simulink model "mocp_simulink_block"  (R2016b)
settings: Solver=ode45  StartTime=0.0  StopTime=0.1  RelTol=1e-3
values from neighbouring files (symbols this model uses):
  ignore_inits = 0    [main_mocp_simulink.m]
  lbu_all = bu_fact * lbu_all    [main_mocp_simulink.m]
  lbx_all = [repmat(phase_1.constraints.lbx, N_list(1)-1, 1) ... (first row only)    [main_mocp_simulink.m]
  lh_all = [repmat(phase_1.constraints.lh, N_list(1)-1, 1) ... (first row only)    [main_mocp_simulink.m]
  pi_init = 0 * pi_traj    [main_mocp_simulink.m]
  reset_solver = 0    [main_mocp_simulink.m]
  u_init = 0 * u_traj    [main_mocp_simulink.m]
  ubu_all = bu_fact * ubu_all    [main_mocp_simulink.m]
  ubx_all = [repmat(phase_1.constraints.ubx, N_list(1)-1, 1) ... (first row only)    [main_mocp_simulink.m]
  uh_all = [repmat(phase_1.constraints.uh, N_list(1)-1, 1) ... (first row only)    [main_mocp_simulink.m]
  x0_original = phase_1.constraints.x0    [main_mocp_simulink.m]
  x_init = 0 * x_traj    [main_mocp_simulink.m]    (also in main_multiphase_ocp.m = [repmat(x0, 1, N_list(1)+N_list(2)) repmat(x0(1), 1, N_list()
settings Model: Creator=oj  LastModifiedBy=oj
settings DataIOCC: SaveFormat=StructureWithTime  ReturnWorkspaceOutputs=on
settings OptimizationCC: LifeSpan=inf
settings DebuggingCC: FcnCallInpInsideContextMsg=warning  SFExecutionAtInitializationDiag=none
settings HardwareCC: ProdBitPerSizeT=32  ProdBitPerPtrDiffT=32  ProdWordSize=32  ProdHWDeviceType=Specified
settings ModelReferenceCC: EnableRefExpFcnMdlSchedulingChecks=off
settings SFSimCC: SimUseLocalCustomCode=on
settings RTWCC: RTWUseLocalCustomCode=on

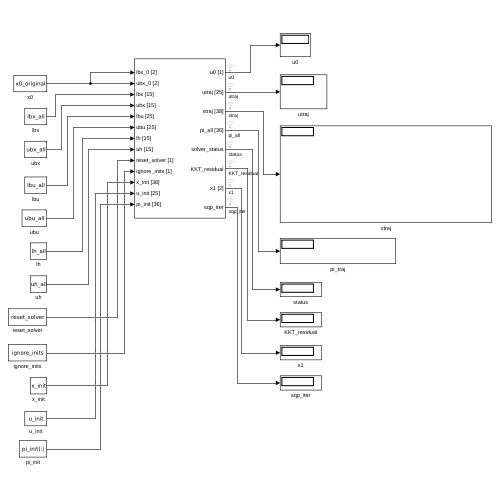
[thumbnail: Simulink's stored preview of the top-level diagram]
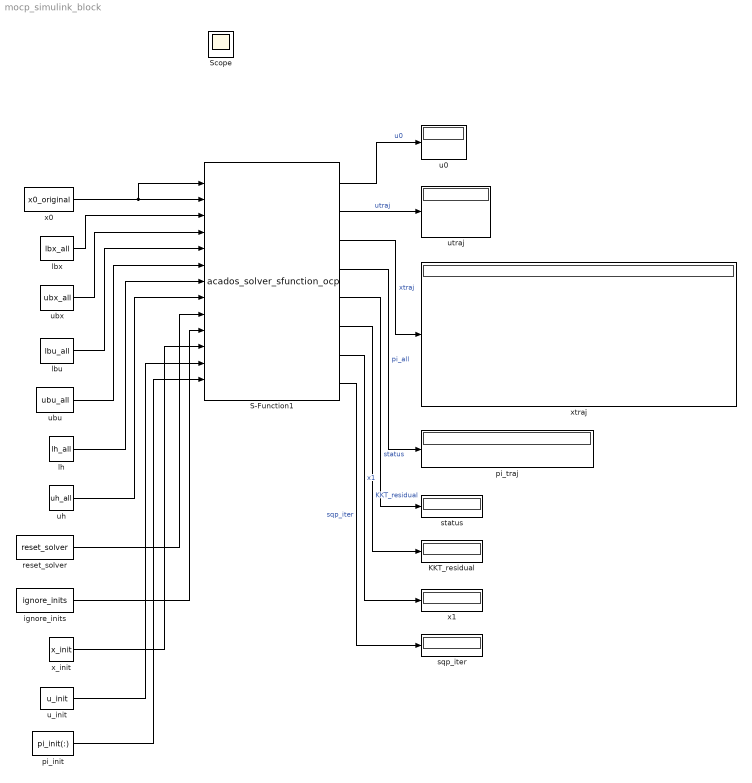
== system mocp_simulink_block ==
  KKT_residual : Display
  S-Function1 : S-Function  FunctionName=acados_solver_sfunction_ocp  SFunctionDeploymentMode=off  EnableBusSupport=off
      mask Display:
      | global sfun_input_names sfun_output_names
      | for i = 1:length(sfun_input_names)
      | 	port_label('input', i, sfun_input_names{i})
      | end
      | for i = 1:length(sfun_output_names)
      | 	port_label('output', i, sfun_output_names{i})
      | end
  ignore_inits : Constant  Value=ignore_inits
  lbu : Constant  Value=lbu_all
  lbx : Constant  Value=lbx_all
  lh : Constant  Value=lh_all
  pi_init : Constant  Value=pi_init(:)
  pi_traj : Display
  reset_solver : Constant  Value=reset_solver
  sqp_iter : Display
  status : Display
  u0 : Display
  u_init : Constant  Value=u_init
  ubu : Constant  Value=ubu_all
  ubx : Constant  Value=ubx_all
  uh : Constant  Value=uh_all
  utraj : Display
  x0 : Constant  Value=x0_original
  x1 : Display
  x_init : Constant  Value=x_init
  xtraj : Display
  Scope : Scope
  wires:
  S-Function1/8 -> sqp_iter/1  "sqp_iter"
  S-Function1/7 -> x1/1  "x1"
  S-Function1/6 -> KKT_residual/1  "KKT_residual"
  S-Function1/2 -> utraj/1  "utraj"
  S-Function1/5 -> status/1  "status"
  x0/1 -> S-Function1/1, S-Function1/2
  lbx/1 -> S-Function1/3
  ubx/1 -> S-Function1/4
  lh/1 -> S-Function1/7
  pi_init/1 -> S-Function1/13
  lbu/1 -> S-Function1/5
  reset_solver/1 -> S-Function1/9
  S-Function1/4 -> pi_traj/1  "pi_all"
  x_init/1 -> S-Function1/11
  S-Function1/3 -> xtraj/1  "xtraj"
  ubu/1 -> S-Function1/6
  S-Function1/1 -> u0/1  "u0"
  uh/1 -> S-Function1/8
  ignore_inits/1 -> S-Function1/10
  u_init/1 -> S-Function1/12
